simulink library "sfReuseStatesLibrary"  (R2025b)
settings: Solver=VariableStepAuto  StartTime=0.0  StopTime=10.0  RelTol=1e-3
settings Model: Creator=The MathWorks, Inc.  LastModifiedBy=The MathWorks, Inc.
settings SolverCC: AlgebraicLoopSolver=TrustRegion
settings OptimizationCC: ReuseModelBlockBuffer=off
settings DebuggingCC: UnconnectedInputMsg=warning  UnconnectedOutputMsg=warning  UnconnectedLineMsg=warning  SymbolicDimsDataTypeCodeGenerationDiagnostic=none
settings ModelReferenceCC: EnableRefExpFcnMdlSchedulingChecks=on
settings RTWCC: GPUComputeCapability=3.5

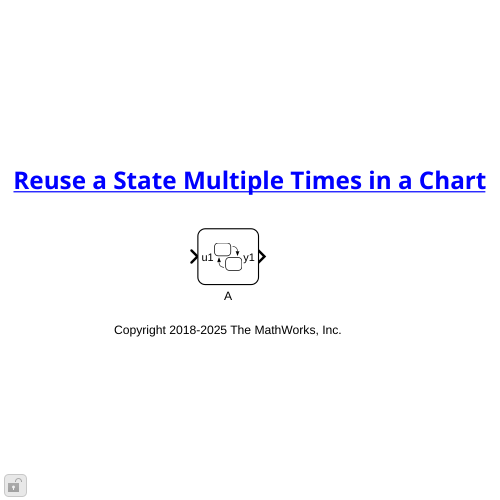
[thumbnail: Simulink's stored preview of the top-level diagram]
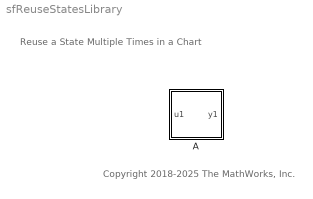
== system sfReuseStatesLibrary ==
  note: Copyright 2018-2025 The MathWorks, Inc.
  note: Reuse a State Multiple Times in a Chart
  A : Stateflow chart  BlockKeywords=__PRM__SERIALIZED__DATA__:Stateflow Chart,Stateflow Diagram  TreatAsAtomicUnit=on

== stateflow chart sfReuseStatesLibrary/A ==
  state Pos
    entry: y1 = 1;
  state Neg
    entry: y1 = -1;
  (default) -> Pos [order 1] : [u1 > 0]
  (default) -> Neg [order 2]
  Pos -> Neg : [u1 < 0]
  Neg -> Pos : [u1 > 0]
  data: u1 input; y1 output double
